simulink model "proyectoControl"  (R2025b)
settings: Solver=ode4  StartTime=0.0  StopTime=15  FixedStep=0.01  RelTol=1e-3
undefined symbols (not defined in the file or in its folder): dspblkCoreblockFVToolHelper, gcbh
settings Model: Creator=kenne  LastModifiedBy=kenne

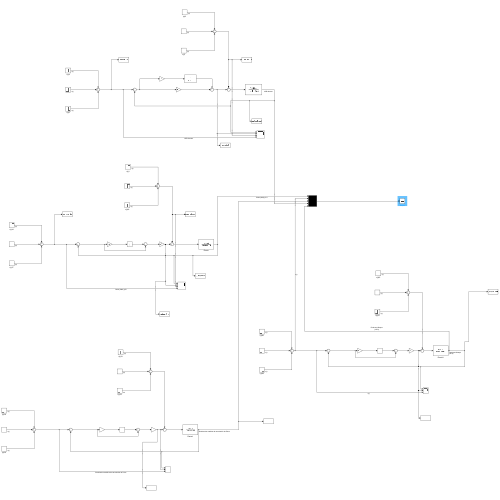
[thumbnail: Simulink's stored preview of the top-level diagram]
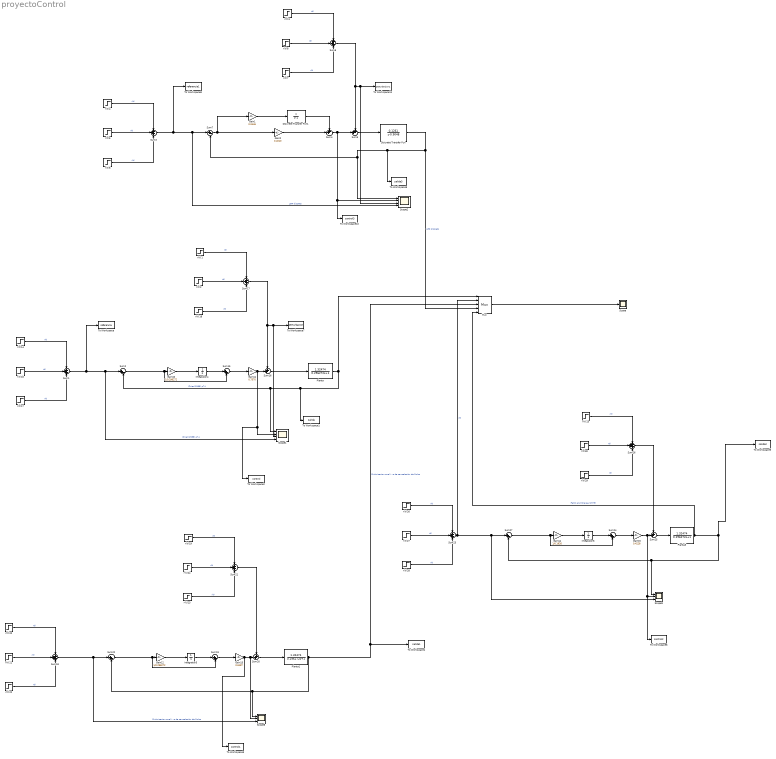
== system proyectoControl ==
  Discrete Transfer Fcn : DiscreteTransferFcn  LoadFcn=dspblkCoreblockFVToolHelper(gcbh,'load');  Numerator=[0.1261]  Denominator=[1 -0.9048]
      settings: CopyFcn=dspblkCoreblockFVToolHelper(gcbh,'copy');  DeleteFcn=dspblkCoreblockFVToolHelper(gcbh,'close');  ModelCloseFcn=dspblkCoreblockFVToolHelper(gcbh,'close');  PreSaveFcn=dspblkCoreblockFVToolHelper(gcbh,'presave');  PostSaveFcn=dspblkCoreblockFVToolHelper(gcbh,'postsave');  CloseFcn=dspblkCoreblockFVToolHelper(gcbh,'close');
  Discrete Transfer Fcn1 : DiscreteTransferFcn  LoadFcn=dspblkCoreblockFVToolHelper(gcbh,'load');  Numerator=[1 0]  Denominator=[1 -1]
      settings: CopyFcn=dspblkCoreblockFVToolHelper(gcbh,'copy');  DeleteFcn=dspblkCoreblockFVToolHelper(gcbh,'close');  ModelCloseFcn=dspblkCoreblockFVToolHelper(gcbh,'close');  PreSaveFcn=dspblkCoreblockFVToolHelper(gcbh,'presave');  PostSaveFcn=dspblkCoreblockFVToolHelper(gcbh,'postsave');  CloseFcn=dspblkCoreblockFVToolHelper(gcbh,'close');
  Gain1 : Gain  Gain=0.0446
  Gain10 : Gain  Gain=1/0.296272
  Gain11 : Gain  Gain=0.7570
  Gain12 : Gain  Gain=1/0.296272
  Gain13 : Gain  Gain=0.6187
  Gain14 : Gain  Gain=1/0.1926
  Gain15 : Gain  Gain=0.4228
  Gain2 : Gain  Gain=0.4010
  Integrator4 : Integrator
  Integrator5 : Integrator
  Integrator6 : Integrator
  Mux : Mux  Inputs=5
  Planta : TransferFcn  Numerator=[0 1.32474]  Denominator=[0.296272 1]
  Planta1 : TransferFcn  Numerator=[0 1.32474]  Denominator=[0.296272 1]
  Planta3 : TransferFcn  Numerator=[0 1.32474]  Denominator=[0.296272 1]
  Scope : Scope
      settings: ActiveDisplayYMinimum=-13.451696560194303  ActiveDisplayYMaximum=121.06526904174876  DataLoggingVariableName=ScopeData2
  Scope1 : Scope  NumInputPorts=4
      settings: ActiveDisplayYMinimum=-25.413301193862964  ActiveDisplayYMaximum=155.27192535965935
  Scope2 : Scope  NumInputPorts=4
      settings: ActiveDisplayYMinimum=-14.939706147554354  ActiveDisplayYMaximum=150.94952006506713  DataLoggingVariableName=ScopeData3
  Scope8 : Scope  NumInputPorts=3
      settings: ActiveDisplayYMinimum=-41.83171933312574  ActiveDisplayYMaximum=155.86406904319611
  Scope9 : Scope  NumInputPorts=3
      settings: ActiveDisplayYMinimum=-30.05398305487391  ActiveDisplayYMaximum=195.02503896499778  DataLoggingVariableName=ScopeData8
  Sum{1,3,6,17..18,21,23,26} (8 alike) : Sum  Inputs=+++
  Sum15 : Sum  Inputs=|++
  Sum{4..5,16,20,25} (5 alike) : Sum  Inputs=++|
  Sum19 : Sum  Inputs=|++
  Sum{2,7,22,27} (4 alike) : Sum  Inputs=|+-
  Sum24 : Sum  Inputs=|++
  To Workspace : ToWorkspace  VariableName=referencia  SaveFormat=Timeseries  SampleTime=-1
  To Workspace1 : ToWorkspace  VariableName=salida  SaveFormat=Timeseries  SampleTime=-1
  To Workspace10 : ToWorkspace  VariableName=control3  SaveFormat=Timeseries  SampleTime=-1
  To Workspace11 : ToWorkspace  VariableName=perturbacion1  SaveFormat=Timeseries  SampleTime=-1
  To Workspace2 : ToWorkspace  VariableName=control  SaveFormat=Timeseries  SampleTime=-1
  To Workspace3 : ToWorkspace  VariableName=control1  SaveFormat=Timeseries  SampleTime=-1
  To Workspace4 : ToWorkspace  VariableName=salida1  SaveFormat=Timeseries  SampleTime=-1
  To Workspace5 : ToWorkspace  VariableName=salida2  SaveFormat=Timeseries  SampleTime=-1
  To Workspace6 : ToWorkspace  VariableName=control2  SaveFormat=Timeseries  SampleTime=-1
  To Workspace7 : ToWorkspace  VariableName=perturbacion  SaveFormat=Timeseries  SampleTime=-1
  To Workspace8 : ToWorkspace  VariableName=referencia1  SaveFormat=Timeseries  SampleTime=-1
  To Workspace9 : ToWorkspace  VariableName=salida3  SaveFormat=Timeseries  SampleTime=-1
  r(t)1 : Step  Time=10  After=10  SampleTime=0
  r(t){4,14,20,26} (4 alike) : Step  Time=0  After=90  SampleTime=0
  r(t){5,16,21,27} (4 alike) : Step  Time=30  After=30  SampleTime=0
  r(t){6,17,22,28} (4 alike) : Step  Time=50  After=-30  SampleTime=0
  r(t)18 : Step  Time=60  After=10  SampleTime=0
  r(t)19 : Step  Time=10  After=30  SampleTime=0
  r(t)2 : Step  Time=40  After=10  SampleTime=0
  r(t)23 : Step  Time=60  After=30  SampleTime=0
  r(t)24 : Step  Time=40  After=30  SampleTime=0
  r(t)25 : Step  Time=10  After=30  SampleTime=0
  r(t)29 : Step  Time=60  After=30  SampleTime=0
  r(t)3 : Step  Time=10  After=10  SampleTime=0
  r(t)30 : Step  Time=40  After=30  SampleTime=0
  r(t)7 : Step  Time=60  After=10  SampleTime=0
  r(t)8 : Step  Time=40  After=10  SampleTime=0
  wires:
  Sum1/1 -> To Workspace/1, Scope1/4, Sum2/1  "Chien(1988) p74"
  r(t)16/1 -> Sum1/2  "r(t)"
  r(t)14/1 -> Sum1/1  "r(t)"
  r(t)17/1 -> Sum1/3  "r(t)"
  Gain10/1 -> Integrator4/1
  Sum2/1 -> Sum15/2, Gain10/1
  Integrator4/1 -> Sum15/1
  Sum15/1 -> Gain11/1
  Gain11/1 -> To Workspace2/1, Scope1/2, Sum16/2
  r(t)1/1 -> Sum17/1  "r(t)"
  r(t)2/1 -> Sum17/2  "r(t)"
  Sum17/1 -> Scope1/3, To Workspace7/1, Sum16/1
  Sum16/1 -> Planta/1
  Planta/1 -> To Workspace1/1, Scope1/1, Sum2/2, Mux/1  "Chien(1988) p74"
  Gain12/1 -> Integrator5/1
  Integrator5/1 -> Sum19/1
  Sum19/1 -> Gain13/1
  Sum22/1 -> Sum19/2, Gain12/1
  Sum21/1 -> Sum20/1
  r(t)24/1 -> Sum21/2  "r(t)"
  r(t)19/1 -> Sum21/1  "r(t)"
  Gain13/1 -> To Workspace3/1, Scope8/2, Sum20/2
  r(t)21/1 -> Sum18/2  "r(t)"
  Sum18/1 -> Scope8/3, Sum22/1  "Sintinizacion analítica de cancelación de Polos"
  r(t)23/1 -> Sum21/3  "r(t)"
  r(t)20/1 -> Sum18/1  "r(t)"
  r(t)22/1 -> Sum18/3  "r(t)"
  r(t)27/1 -> Sum23/2  "r(t)"
  r(t)26/1 -> Sum23/1  "r(t)"
  Sum23/1 -> Mux/2, Scope9/3, Sum27/1  "r(t)"
  r(t)28/1 -> Sum23/3  "r(t)"
  r(t)25/1 -> Sum26/1  "r(t)"
  r(t)30/1 -> Sum26/2  "r(t)"
  Sum27/1 -> Sum24/2, Gain14/1
  Sum24/1 -> Gain15/1
  Gain14/1 -> Integrator6/1
  Sum26/1 -> Sum25/1
  Gain15/1 -> Scope9/2, To Workspace6/1, Sum25/2
  Integrator6/1 -> Sum24/1
  r(t)29/1 -> Sum26/3  "r(t)"
  r(t)18/1 -> Sum17/3  "r(t)"
  Sum20/1 -> Planta1/1
  Planta1/1 -> Sum22/2, Scope8/1, To Workspace4/1, Mux/3  "Sintinizacion analítica de cancelación de Polos"
  Sum25/1 -> Planta3/1
  Planta3/1 -> Mux/5, To Workspace5/1, Scope9/1, Sum27/2  "Fertik and Sharpe (1979)"
  Mux/1 -> Scope/1
  Discrete Transfer Fcn/1 -> Mux/4, Scope2/1, Sum7/2, To Workspace9/1  "LGR discreto"
  r(t)8/1 -> Sum6/2  "r(t)"
  Sum5/1 -> Discrete Transfer Fcn/1
  Sum6/1 -> Scope2/3, To Workspace11/1, Sum5/1
  r(t)7/1 -> Sum6/3  "r(t)"
  r(t)6/1 -> Sum3/3  "r(t)"
  r(t)3/1 -> Sum6/1  "r(t)"
  Sum3/1 -> To Workspace8/1, Sum7/1, Scope2/4  "LGR discreto"
  r(t)4/1 -> Sum3/1  "r(t)"
  Sum7/1 -> Gain2/1, Gain1/1
  r(t)5/1 -> Sum3/2  "r(t)"
  Discrete Transfer Fcn1/1 -> Sum4/1
  Sum4/1 -> Sum5/2, Scope2/2, To Workspace10/1
  Gain1/1 -> Discrete Transfer Fcn1/1
  Gain2/1 -> Sum4/2
